simulink model "pid_board_tb_analog"  (R2024b)
settings: Solver=ode4  StartTime=0.0  StopTime=pbsim.t_stop  FixedStep=pcb.sim_dt  RelTol=1e-3
PostLoadFcn:
  | pbdir_ = fileparts(get_param('pid_board_tb_analog', 'FileName')); if ~exist('pcb', 'var'), run(fullfile(pbdir_, 'pid_board_params.m')); end; clear pbdir_
settings Model: Creator=doubi  LastModifiedBy=doubi

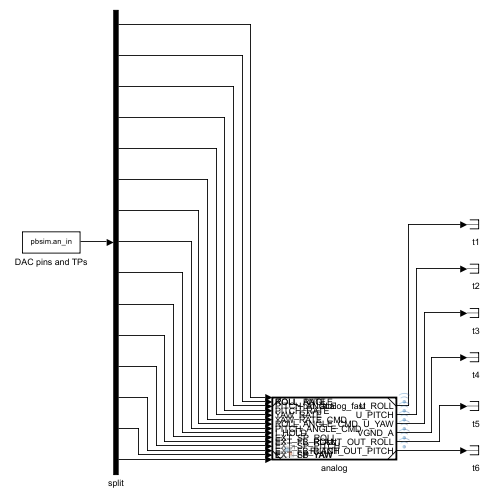
[thumbnail: Simulink's stored preview of the top-level diagram]
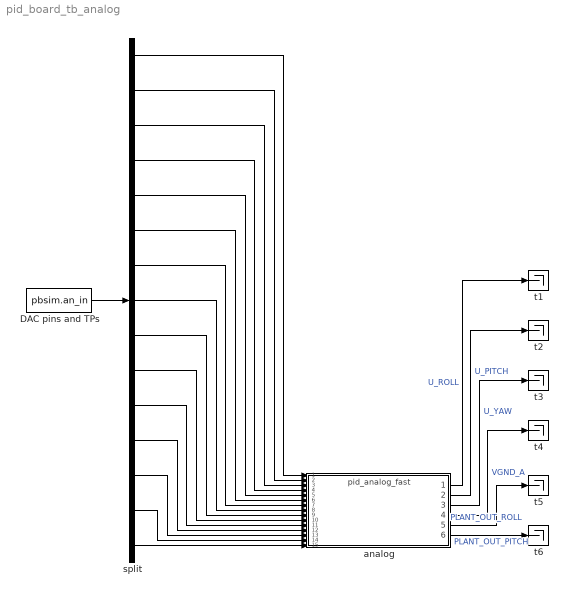
== system pid_board_tb_analog ==
  DAC pins and TPs : FromWorkspace  VariableName=pbsim.an_in  OutputAfterFinalValue=Holding final value
  analog : ModelReference  ModelNameDialog=pid_analog_fast  SimulationMode=Normal  ModelReferenceVersion=1.1
  split : Demux  Outputs=15
  t{1..6} (6 alike) : Terminator
  wires:
  split/14 -> analog/14
  split/6 -> analog/6
  analog/3 -> t3/1  "U_YAW"
  split/4 -> analog/4
  split/12 -> analog/12
  split/3 -> analog/3
  split/8 -> analog/8
  split/2 -> analog/2
  DAC pins and TPs/1 -> split/1
  split/1 -> analog/1
  split/7 -> analog/7
  split/5 -> analog/5
  split/9 -> analog/9
  split/10 -> analog/10
  split/11 -> analog/11
  split/13 -> analog/13
  split/15 -> analog/15
  analog/1 -> t1/1  "U_ROLL"
  analog/2 -> t2/1  "U_PITCH"
  analog/4 -> t4/1  "VGND_A"
  analog/5 -> t5/1  "PLANT_OUT_ROLL"
  analog/6 -> t6/1  "PLANT_OUT_PITCH"
